simulink model "skf_1x2x2"  (R2023a)
settings: Solver=ode1be  StartTime=0.0  StopTime=40  FixedStep=Ts  RelTol=1e-3
values from neighbouring files (symbols this model uses):
  F_np = eye(M)    [Initialization_fxKalman.m]
  m = 4    [Initialization_fxKalman.m]
  M = 70    [Initialization_1x1x1.m]    (also in Initialization_1x2x2.m = 150; Initialization_fxKalman.m = 200; Initialization_path_estimation.m = 200)
  mu1 = 2    [Initialization_1x1x1.m]    (also in Initialization_1x2x2.m = 10; Initialization_fxKalman.m = 0.5)
  mu2 = 1    [Initialization_1x1x1.m]    (also in Initialization_1x2x2.m; Initialization_fxKalman.m = 0.1)
  n = 1    [Initialization_1x1x1.m]    (also in Initialization_1x2x2.m = 4; Initialization_fxKalman.m = zeros(M,C))
  P = (5e-6)*eye(N)    [Initialization_1x1x1.m]    (also in Initialization_1x2x2.m; Initialization_fxKalman.m = (5e-6)*eye(M))
  Q_np = sigma_q^2*eye(M)    [Initialization_fxKalman.m]
  R_np = (sigma_r^2)*eye(K*N)    [Initialization_fxKalman.m]
  Ts = 1/fs    (= 0.001)    [Initialization_1x1x1.m]    (also in Initialization_1x2x2.m; Initialization_fxKalman.m; Initialization_path_estimation.m)
undefined symbols (not defined in the file or in its folder): S11, S12, S21, S22
libraries: simulink x4, speedgoatlib_IO104 x3, matrix_library x2, dspsrcs4 x1
settings Model: Creator=Tamida  LastModifiedBy=tislam
settings SolverCC: ConcurrentTasks=on  PositivePriorityOrder=on
settings DataIOCC: MaxDataPoints=1
settings OptimizationCC: BlockReduction=off  OptimizeBlockIOStorage=off  ReuseModelBlockBuffer=off
settings DebuggingCC: TasksWithSamePriorityMsg=none
settings HardwareCC: ProdBitPerLong=64  ProdLongLongMode=on  ProdHWDeviceType=Intel->x86-64 (Linux 64)
settings RTWCC: Description=Simulink Real-Time  SystemTargetFile=slrealtime.tlc  TemplateMakefile=slrealtime_default_tmf  Toolchain=Simulink Real-Time Toolchain  BuildConfiguration=Faster Runs  CodeExecutionProfiling=on  TargetLang=C++

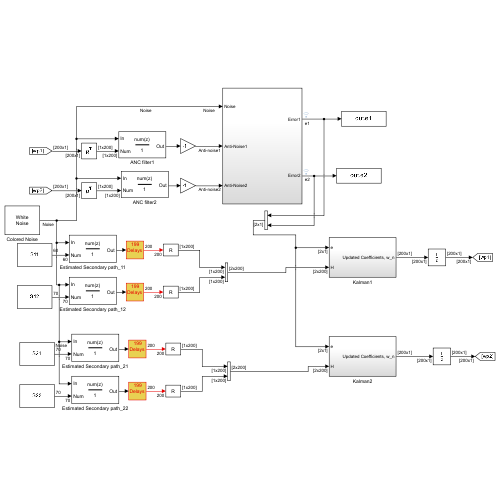
[thumbnail: Simulink's stored preview of the top-level diagram]
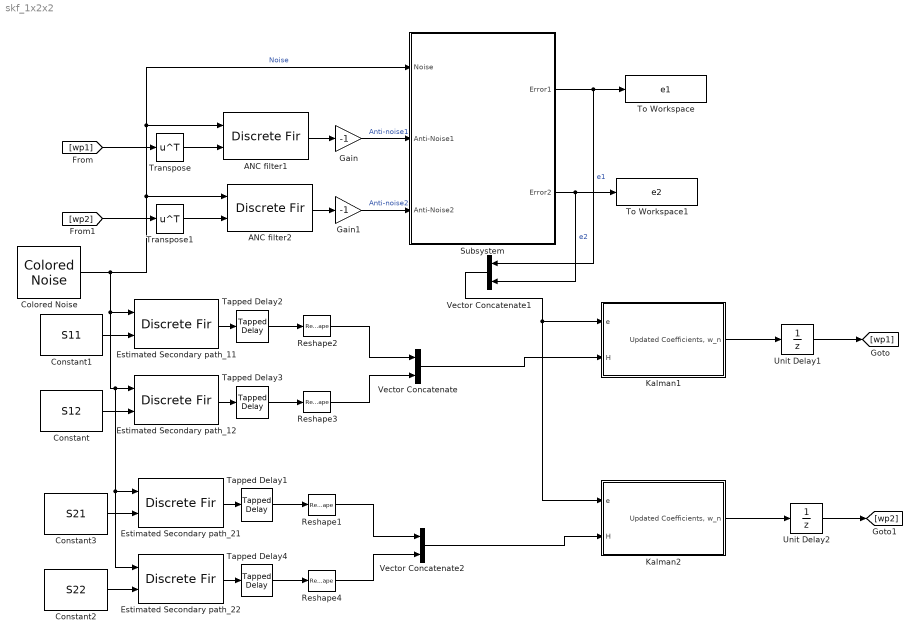
== system skf_1x2x2 ==
  ANC filter1 : DiscreteFir  CoefSource=Input port
      settings: InputPortMap=u0,u1
  ANC filter2 : DiscreteFir  CoefSource=Input port
      settings: InputPortMap=u0,u1
  Colored Noise : dspsrcs4/Colored Noise  Color=white  InverseFrequencyPower=1  BoundedOutput=on  NumChannels=1  OutputDataType=double  SamplesPerFrame=1  SampleTime=Ts  RandomStream=mt19937ar with seed  Seed=67  SimulateUsing=Interpreted execution
      settings: LibrarySourceBlock=audiosources/Colored Noise
  Constant : Constant  Value=S12  SampleTime=-1
  Constant1 : Constant  Value=S11  SampleTime=-1
  Constant2 : Constant  Value=S22  SampleTime=-1
  Constant3 : Constant  Value=S21  SampleTime=-1
  Estimated Secondary path_{11..12,21..22} (4 alike) : DiscreteFir  CoefSource=Input port  Coefficients=[-1.6 -0.6 -.25 0.4 -1.5 0.4 -1.2 0.07 0.6 0.3]
      settings: InputPortMap=u0,u1
  Gain : Gain  Gain=-1
  Gain1 : Gain  Gain=-1
  Kalman1 : Subsystem
  Kalman2 : Subsystem
  Reshape{1..4} (4 alike) : Reshape  OutputDimensionality=Customize  OutputDimensions=[1,M]
  Subsystem : Subsystem
  Tapped Delay{1..4} (4 alike) : simulink/Discrete/Tapped Delay  vinit=0.0  samptime=-1  NumDelays=M-1  DelayOrder=Newest  includeCurrent=on
  To Workspace : ToWorkspace  VariableName=e1  SaveFormat=Structure With Time  SampleTime=-1
  To Workspace1 : ToWorkspace  VariableName=e2  SaveFormat=Structure With Time  SampleTime=-1
  Transpose : Math  Operator=transpose
  Transpose1 : Math  Operator=transpose
  Unit Delay1 : UnitDelay  SampleTime=Ts  HasFrameUpgradeWarning=on
  Unit Delay2 : UnitDelay  SampleTime=Ts  HasFrameUpgradeWarning=on
  Vector Concatenate : Concatenate  Mode=Multidimensional array
  Vector Concatenate1 : Concatenate  Mode=Multidimensional array
  Vector Concatenate2 : Concatenate  Mode=Multidimensional array
  wires:
  [wp1] -> Transpose/1
  ANC filter1/1 -> Gain/1
  Constant/1 -> Estimated Secondary path_12/2
  Gain/1 -> Subsystem/2(Anti-Noise1)  "Anti-noise1"
  Subsystem/1(Error1) -> To Workspace/1, Vector Concatenate1/1  "e1"
  Unit Delay1/1 -> [wp1]
  Vector Concatenate/1 -> Kalman1/2(H)
  Kalman1/1("Updated Coefficients, w_n") -> Unit Delay1/1
  Subsystem/2(Error2) -> To Workspace1/1, Vector Concatenate1/2  "e2"
  Constant1/1 -> Estimated Secondary path_11/2
  Tapped Delay2/1 -> Reshape2/1
  Tapped Delay3/1 -> Reshape3/1
  Estimated Secondary path_12/1 -> Tapped Delay3/1
  Reshape3/1 -> Vector Concatenate/2
  Estimated Secondary path_11/1 -> Tapped Delay2/1
  Reshape2/1 -> Vector Concatenate/1
  Tapped Delay1/1 -> Reshape1/1
  Estimated Secondary path_22/1 -> Tapped Delay4/1
  Tapped Delay4/1 -> Reshape4/1
  Constant3/1 -> Estimated Secondary path_21/2
  Reshape1/1 -> Vector Concatenate2/1
  Reshape4/1 -> Vector Concatenate2/2
  Constant2/1 -> Estimated Secondary path_22/2
  Estimated Secondary path_21/1 -> Tapped Delay1/1
  ANC filter2/1 -> Gain1/1
  [wp2] -> Transpose1/1
  Colored Noise/1 -> Subsystem/1("Noise "), ANC filter1/1, ANC filter2/1, Estimated Secondary path_11/1, Estimated Secondary path_21/1, Estimated Secondary path_22/1, Estimated Secondary path_12/1  "Noise"
  Gain1/1 -> Subsystem/3(Anti-Noise2)  "Anti-noise2"
  Vector Concatenate2/1 -> Kalman2/2(H)
  Unit Delay2/1 -> [wp2]
  Vector Concatenate1/1 -> Kalman2/1(e), Kalman1/1(e)
  Kalman2/1("Updated Coefficients, w_n") -> Unit Delay2/1
  Transpose/1 -> ANC filter1/2
  Transpose1/1 -> ANC filter2/2

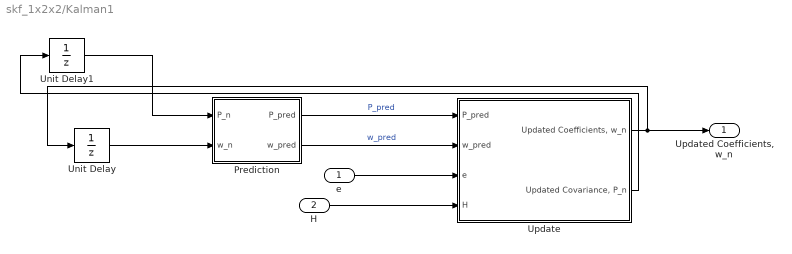
== system skf_1x2x2/Kalman1 ==
  e : Inport
  H : Inport  Port=2
  Prediction : Subsystem
  Unit Delay : UnitDelay  InitialCondition=n  SampleTime=Ts  HasFrameUpgradeWarning=on
  Unit Delay1 : UnitDelay  InitialCondition=P  SampleTime=Ts  HasFrameUpgradeWarning=on
  Update : Subsystem
  "Updated Coefficients, w_n" : Outport
  wires:
  Prediction/1(P_pred) -> Update/1(P_pred)  "P_pred"
  H/1 -> Update/4(H)
  e/1 -> Update/3(e)
  Prediction/2(w_pred) -> Update/2(w_pred)  "w_pred"
  Update/2("Updated Covariance, P_n") -> Unit Delay1/1
  Update/1("Updated Coefficients, w_n") -> "Updated Coefficients, w_n"/1, Unit Delay/1
  Unit Delay/1 -> Prediction/2(w_n)
  Unit Delay1/1 -> Prediction/1(P_n)

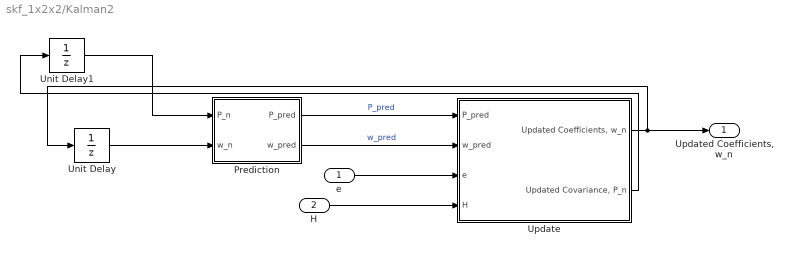
== system skf_1x2x2/Kalman2 ==
  e : Inport
  H : Inport  Port=2
  Prediction : Subsystem
  Unit Delay : UnitDelay  InitialCondition=n  SampleTime=Ts  HasFrameUpgradeWarning=on
  Unit Delay1 : UnitDelay  InitialCondition=P  SampleTime=Ts  HasFrameUpgradeWarning=on
  Update : Subsystem
  "Updated Coefficients, w_n" : Outport
  wires:
  Unit Delay1/1 -> Prediction/1(P_n)
  Unit Delay/1 -> Prediction/2(w_n)
  Update/1("Updated Coefficients, w_n") -> Unit Delay/1, "Updated Coefficients, w_n"/1
  Update/2("Updated Covariance, P_n") -> Unit Delay1/1
  Prediction/2(w_pred) -> Update/2(w_pred)  "w_pred"
  e/1 -> Update/3(e)
  H/1 -> Update/4(H)
  Prediction/1(P_pred) -> Update/1(P_pred)  "P_pred"

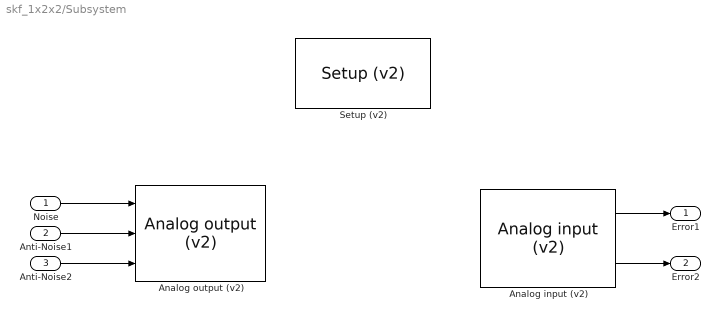
== system skf_1x2x2/Subsystem ==
  "Noise " : Inport
  Anti-Noise1 : Inport  Port=2
  Anti-Noise2 : Inport  Port=3
  "Analog input (v2) " : speedgoatlib_IO104/Analog input (v2)   parModuleId=1  parTs=Ts  parPciSlot=-1  parAdChannels=[7,8]  parAdChannelsSorted=[7,8]  parAdRange1=+-2.5V  parAdRange2=+-2.5V  parAdCoupling=Differential  parAdFrameSize=1  parAdUseTrigger=off  parAdClockInitiator=Initiator  parAdSampleTime=1.000000000e-03  parTriggerInitiator=Initiator  parTriggerRate=4.161015625e-01
      settings: SourceProductName=Simulink Real-Time: Speedgoat I/O Blockset
  "Analog output (v2) " : speedgoatlib_IO104/Analog output (v2)   parModuleId=1  parTs=Ts  parPciSlot=-1  parDaSimultaneous=on  parDaChannels=[2,3,4]  parDaChannelsSorted=[2,3,4]  parDaInitValue=[0,0,0]  parDaReset=[1,1,1]  parDaRange=+-2.5V  parDaFrameSize=1  parDaUseTrigger=off  parDaClockInitiator=Initiator  parDaSampleTime=1.000000000e-03  parTriggerInitiator=Initiator  parTriggerRate=4.161015625e-01  parAdBlockPresent=1
      settings: SourceProductName=Simulink Real-Time: Speedgoat I/O Blockset
  "Setup (v2) " : speedgoatlib_IO104/Setup (v2)   parPciSlot=-1  parModuleId=1  parTriggerInitiator=Initiator  parTriggerRate=4.161015625e-01  parCalibrate=on  parAdChannels=[7 8]  parAdRange1=+-2.5V  parAdRange2=+-2.5V  parAdCoupling=Differential  parAdUseTrigger=off  parAdFrameSize=1  parAdClockInitiator=Initiator  parAdSampleTime=Ts  parDaSimultaneous=on  parDaChannels=[2 3 4]  parDaChannelsSorted=[2,3,4]  parDaInitValue=[0]  parDaReset=[1]  parDaRange=+-2.5V  parDaUseTrigger=off  parDaFrameSize=1  parDaClockInitiator=Initiator  parDaSampleTime=Ts  parDioByte0Dir=Outputs  parDioByte1Dir=Inputs  parDoChannels=[1:4]  parDoInitValues=[0]  parDoReset=[1]  parDiChannels=[13:16]
      settings: SourceProductName=Simulink Real-Time: Speedgoat I/O Blockset
  Error1 : Outport
  Error2 : Outport  Port=2
  wires:
  "Noise "/1 -> "Analog output (v2) "/1
  "Analog input (v2) "/1 -> Error1/1
  Anti-Noise1/1 -> "Analog output (v2) "/2
  "Analog input (v2) "/2 -> Error2/1
  Anti-Noise2/1 -> "Analog output (v2) "/3

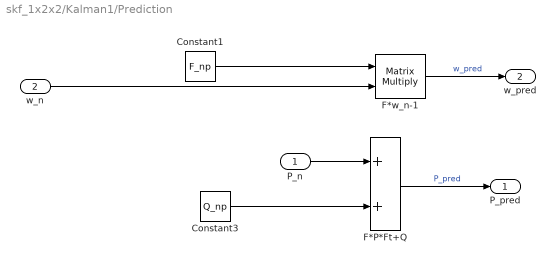
== system skf_1x2x2/Kalman1/Prediction ==
  P_n : Inport
  w_n : Inport  Port=2
  Constant1 : Constant  Value=F_np
  Constant3 : Constant  Value=Q_np
  F*P*Ft+Q : Sum  InputSameDT=on  OutDataTypeStr=Inherit: Inherit via back propagation
  F*w_n-1 : Product  Multiplication=Matrix(*)  InputSameDT=on  OutDataTypeStr=Inherit: Inherit via back propagation
  P_pred : Outport
  w_pred : Outport  Port=2
  wires:
  P_n/1 -> F*P*Ft+Q/1
  Constant3/1 -> F*P*Ft+Q/2
  F*P*Ft+Q/1 -> P_pred/1  "P_pred"
  F*w_n-1/1 -> w_pred/1  "w_pred"
  Constant1/1 -> F*w_n-1/1
  w_n/1 -> F*w_n-1/2

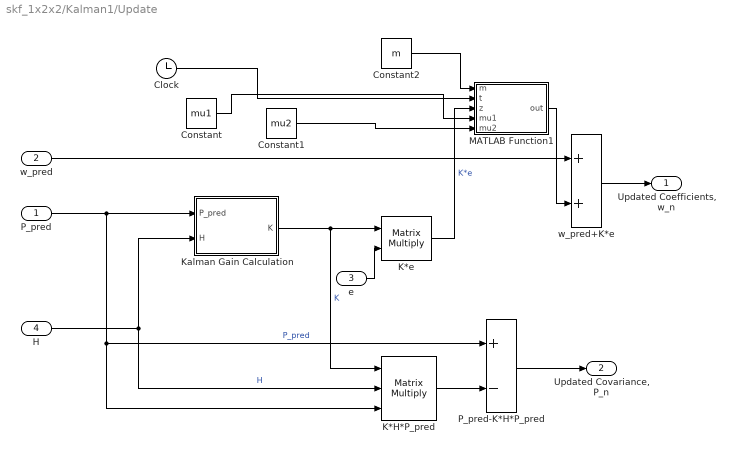
== system skf_1x2x2/Kalman1/Update ==
  P_pred : Inport
  w_pred : Inport  Port=2
  e : Inport  Port=3
  H : Inport  Port=4
  Clock : Clock
  Constant : Constant  Value=mu1
  Constant1 : Constant  Value=mu2
  Constant2 : Constant  Value=m
  K*H*P_pred : Product  Inputs=3  Multiplication=Matrix(*)  InputSameDT=on  OutDataTypeStr=Inherit: Same as first input
  K*e : Product  Multiplication=Matrix(*)  InputSameDT=on  OutDataTypeStr=Inherit: Inherit via back propagation
  Kalman Gain Calculation : Subsystem
  MATLAB Function1 : MATLAB Function  TreatAsAtomicUnit=on
  P_pred-K*H*P_pred : Sum  Inputs=+-  InputSameDT=on  OutDataTypeStr=Inherit: Inherit via back propagation
  w_pred+K*e : Sum  InputSameDT=on  OutDataTypeStr=Inherit: Inherit via back propagation
  "Updated Coefficients, w_n" : Outport
  "Updated Covariance, P_n" : Outport  Port=2
  wires:
  P_pred/1 -> Kalman Gain Calculation/1(P_pred), P_pred-K*H*P_pred/1, K*H*P_pred/3  "P_pred"
  Kalman Gain Calculation/1(K) -> K*H*P_pred/1, K*e/1  "K"
  K*H*P_pred/1 -> P_pred-K*H*P_pred/2
  K*e/1 -> MATLAB Function1/3(z)  "K*e"
  e/1 -> K*e/2
  w_pred+K*e/1 -> "Updated Coefficients, w_n"/1
  H/1 -> Kalman Gain Calculation/2(H), K*H*P_pred/2  "H"
  w_pred/1 -> w_pred+K*e/1
  P_pred-K*H*P_pred/1 -> "Updated Covariance, P_n"/1
  MATLAB Function1/1(out) -> w_pred+K*e/2
  Clock/1 -> MATLAB Function1/2(t)
  Constant/1 -> MATLAB Function1/4(mu1)
  Constant1/1 -> MATLAB Function1/5(mu2)
  Constant2/1 -> MATLAB Function1/1(m)

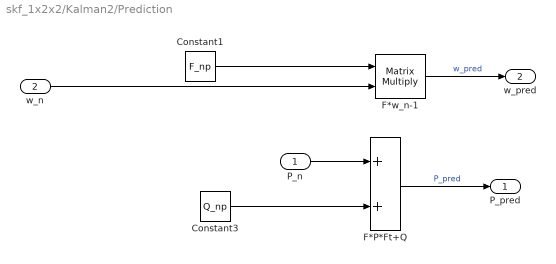
== system skf_1x2x2/Kalman2/Prediction ==
  P_n : Inport
  w_n : Inport  Port=2
  Constant1 : Constant  Value=F_np
  Constant3 : Constant  Value=Q_np
  F*P*Ft+Q : Sum  InputSameDT=on  OutDataTypeStr=Inherit: Inherit via back propagation
  F*w_n-1 : Product  Multiplication=Matrix(*)  InputSameDT=on  OutDataTypeStr=Inherit: Inherit via back propagation
  P_pred : Outport
  w_pred : Outport  Port=2
  wires:
  w_n/1 -> F*w_n-1/2
  Constant1/1 -> F*w_n-1/1
  F*w_n-1/1 -> w_pred/1  "w_pred"
  F*P*Ft+Q/1 -> P_pred/1  "P_pred"
  Constant3/1 -> F*P*Ft+Q/2
  P_n/1 -> F*P*Ft+Q/1

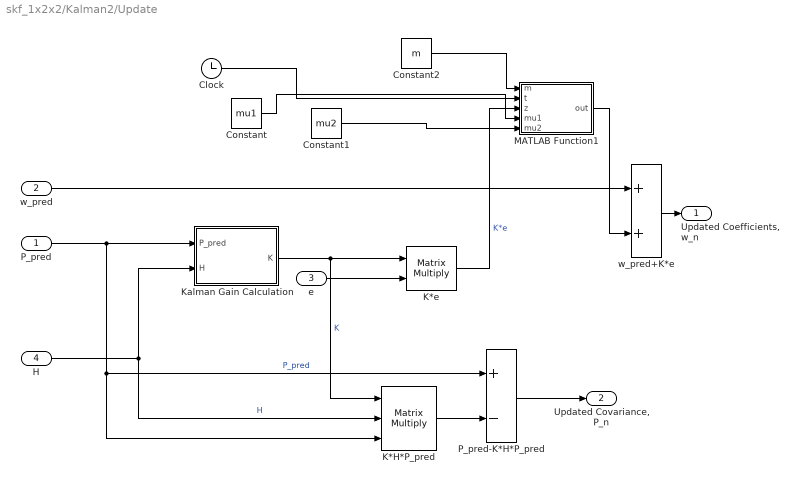
== system skf_1x2x2/Kalman2/Update ==
  P_pred : Inport
  w_pred : Inport  Port=2
  e : Inport  Port=3
  H : Inport  Port=4
  Clock : Clock
  Constant : Constant  Value=mu1
  Constant1 : Constant  Value=mu2
  Constant2 : Constant  Value=m
  K*H*P_pred : Product  Inputs=3  Multiplication=Matrix(*)  InputSameDT=on  OutDataTypeStr=Inherit: Same as first input
  K*e : Product  Multiplication=Matrix(*)  InputSameDT=on  OutDataTypeStr=Inherit: Inherit via back propagation
  Kalman Gain Calculation : Subsystem
  MATLAB Function1 : MATLAB Function  TreatAsAtomicUnit=on
  P_pred-K*H*P_pred : Sum  Inputs=+-  InputSameDT=on  OutDataTypeStr=Inherit: Inherit via back propagation
  w_pred+K*e : Sum  InputSameDT=on  OutDataTypeStr=Inherit: Inherit via back propagation
  "Updated Coefficients, w_n" : Outport
  "Updated Covariance, P_n" : Outport  Port=2
  wires:
  P_pred-K*H*P_pred/1 -> "Updated Covariance, P_n"/1
  w_pred/1 -> w_pred+K*e/1
  H/1 -> K*H*P_pred/2, Kalman Gain Calculation/2(H)  "H"
  w_pred+K*e/1 -> "Updated Coefficients, w_n"/1
  e/1 -> K*e/2
  K*e/1 -> MATLAB Function1/3(z)  "K*e"
  K*H*P_pred/1 -> P_pred-K*H*P_pred/2
  Kalman Gain Calculation/1(K) -> K*H*P_pred/1, K*e/1  "K"
  P_pred/1 -> K*H*P_pred/3, P_pred-K*H*P_pred/1, Kalman Gain Calculation/1(P_pred)  "P_pred"
  MATLAB Function1/1(out) -> w_pred+K*e/2
  Clock/1 -> MATLAB Function1/2(t)
  Constant/1 -> MATLAB Function1/4(mu1)
  Constant1/1 -> MATLAB Function1/5(mu2)
  Constant2/1 -> MATLAB Function1/1(m)

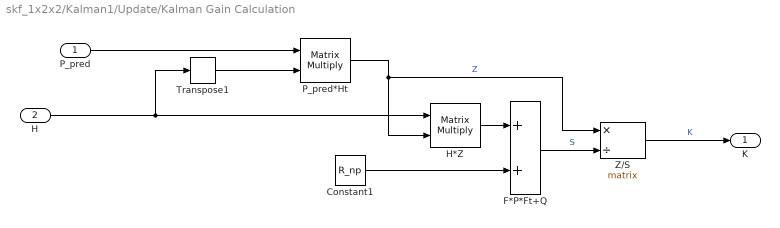
== system skf_1x2x2/Kalman1/Update/Kalman Gain Calculation ==
  P_pred : Inport
  H : Inport  Port=2
  Constant1 : Constant  Value=R_np
  F*P*Ft+Q : Sum  InputSameDT=on  OutDataTypeStr=Inherit: Inherit via back propagation
  H*Z : Product  Multiplication=Matrix(*)  InputSameDT=on  OutDataTypeStr=Inherit: Inherit via back propagation
  P_pred*Ht : Product  Multiplication=Matrix(*)  InputSameDT=on  OutDataTypeStr=Inherit: Inherit via back propagation
  Transpose1 : matrix_library/Transpose
  Z/S : Product  Inputs=*/  Multiplication=Matrix(*)
  K : Outport
  wires:
  P_pred/1 -> P_pred*Ht/1
  Constant1/1 -> F*P*Ft+Q/2
  P_pred*Ht/1 -> Z/S/1, H*Z/2  "Z"
  H/1 -> H*Z/1, Transpose1/1
  F*P*Ft+Q/1 -> Z/S/2  "S"
  H*Z/1 -> F*P*Ft+Q/1
  Transpose1/1 -> P_pred*Ht/2
  Z/S/1 -> K/1  "K"

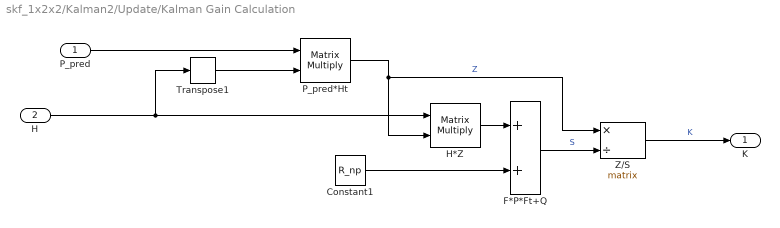
== system skf_1x2x2/Kalman2/Update/Kalman Gain Calculation ==
  P_pred : Inport
  H : Inport  Port=2
  Constant1 : Constant  Value=R_np
  F*P*Ft+Q : Sum  InputSameDT=on  OutDataTypeStr=Inherit: Inherit via back propagation
  H*Z : Product  Multiplication=Matrix(*)  InputSameDT=on  OutDataTypeStr=Inherit: Inherit via back propagation
  P_pred*Ht : Product  Multiplication=Matrix(*)  InputSameDT=on  OutDataTypeStr=Inherit: Inherit via back propagation
  Transpose1 : matrix_library/Transpose
  Z/S : Product  Inputs=*/  Multiplication=Matrix(*)
  K : Outport
  wires:
  Z/S/1 -> K/1  "K"
  Transpose1/1 -> P_pred*Ht/2
  H*Z/1 -> F*P*Ft+Q/1
  F*P*Ft+Q/1 -> Z/S/2  "S"
  H/1 -> Transpose1/1, H*Z/1
  P_pred*Ht/1 -> H*Z/2, Z/S/1  "Z"
  Constant1/1 -> F*P*Ft+Q/2
  P_pred/1 -> P_pred*Ht/1

== matlab function skf_1x2x2/Kalman2/Update/MATLAB Function1 ==
  data: m input; t input; z input; out output; mu1 input; mu2 input
function out = fcn( m, t,z, mu1,mu2)

%#codegen

if t<=m
    out = mu1*z;
else
    out = mu2*z;
end

== matlab function skf_1x2x2/Kalman1/Update/MATLAB Function1 ==
  data: m input; t input; z input; out output; mu1 input; mu2 input
function out = fcn( m, t,z, mu1,mu2)

%#codegen

if t<=m
    out = mu1*z;
else
    out = mu2*z;
end
